simulink model "spikingTest"  (R2026b)
settings: Solver=FixedStepAuto  StopTime=1  FixedStep=0.001
libraries: simulink x1
settings Model: Creator=40129232  LastModifiedBy=Eoin
settings DataIOCC: ReturnWorkspaceOutputs=off
settings OptimizationCC: LifeSpan=inf
settings DebuggingCC: ArithmeticOperatorsInVariantConditions=warning  SFExecutionAtInitializationDiag=none
settings SFSimCC: CustomCodeUndefinedFunction=UseInterfaceOnly  SimUseLocalCustomCode=off
settings RTWCC: DLArmComputeVersion=19.05  RTWUseLocalCustomCode=off
settings CodeAppCC: StateflowObjectComments=on

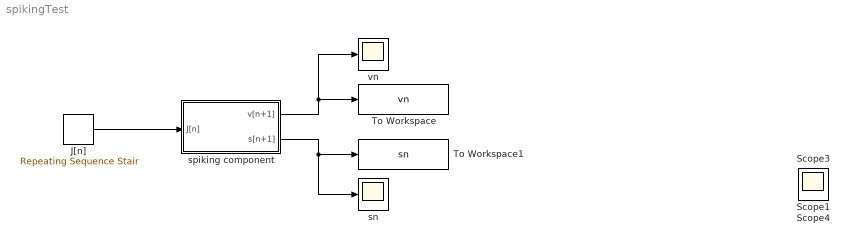
== system spikingTest ==
  J[n] : simulink/Sources/Repeating Sequence Stair  OutValues=[40.37, 52.35, 62.17, 70.19, 76.75].'  tsamp=-1  OutMin=[]  OutMax=[]  OutDataTypeStr=double  OutputDataTypeScalingMode=double  OutDataType=fixdt(0,8)  ConRadixGroup=Best Precision: Vector-wise  OutScaling=2^-12
  To Workspace : ToWorkspace  VariableName=vn  SaveFormat=Timeseries  SampleTime=-1
  To Workspace1 : ToWorkspace  VariableName=sn  SaveFormat=Timeseries  SampleTime=-1
  sn : Scope
      settings: ActiveDisplayYMinimum=-0.12499999999999997  ActiveDisplayYMaximum=1.125
  spiking component : Subsystem
  vn : Scope
      settings: ActiveDisplayYMinimum=-91.151379089259891  ActiveDisplayYMaximum=42.518602095331175  DataLoggingVariableName=ScopeData5
  Scope1 : Scope
      settings: ActiveDisplayYMinimum=-0.24987  ActiveDisplayYMaximum=2.24887
  Scope3 : Scope
      settings: ActiveDisplayYMinimum=-103.72127  ActiveDisplayYMaximum=38.33358  DataLoggingVariableName=ScopeData3
  Scope4 : Scope
      settings: ActiveDisplayYMinimum=-20.75486  ActiveDisplayYMaximum=56.79378  DataLoggingVariableName=ScopeData4
  wires:
  spiking component/1(v[n+1]) -> vn/1, To Workspace/1
  spiking component/2(s[n+1]) -> sn/1, To Workspace1/1
  J[n]/1 -> spiking component/1(J[n])

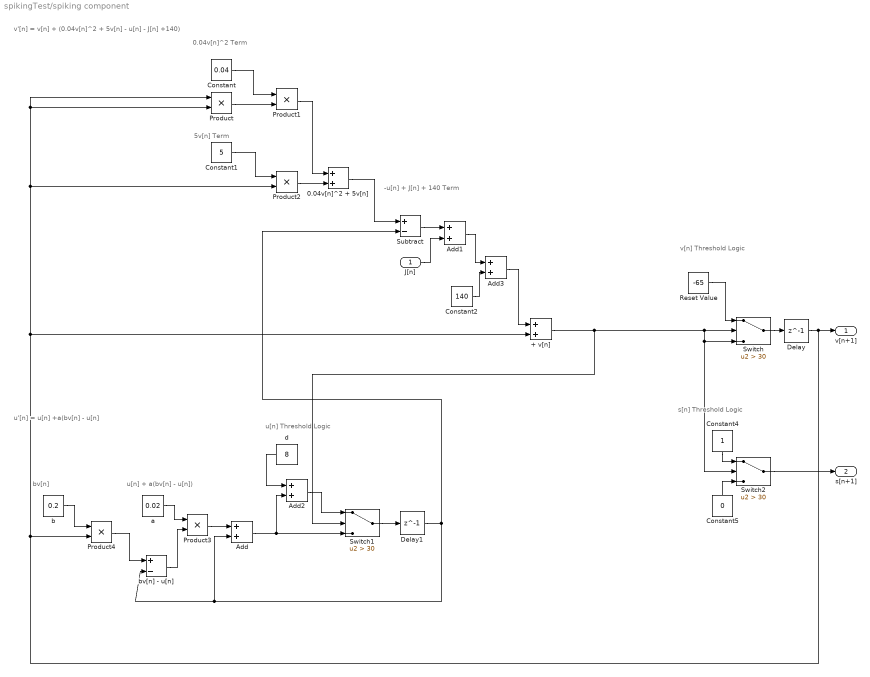
== system spikingTest/spiking component ==
  note: s[n] Threshold Logic
  note: v'[n] = v[n] + (0.04v[n]^2 + 5v[n] - u[n] - J[n] +140)
  note: u'[n] = u[n] +a(bv[n] - u[n]
  note: u[n] Threshold Logic
  note: u[n] + a(bv[n] - u[n])
  note: bv[n]
  note: v[n] Threshold Logic
  note: -u[n] + J[n] + 140 Term
  note: 5v[n] Term
  note: 0.04v[n]^2 Term
  J[n] : Inport  SampleTime=0.001
  + v[n] : Sum
  0.04v[n]^2 + 5v[n] : Sum
  Add{,1..3} (4 alike) : Sum
  Constant : Constant  Value=0.04
  Constant1 : Constant  Value=5
  Constant2 : Constant  Value=140
  Constant4 : Constant
  Constant5 : Constant  Value=0
  Delay : Delay  DelayLength=1  InitialCondition=-65
  Delay1 : Delay  DelayLength=1  InitialCondition=0
  Product{,1..4} (5 alike) : Product
  Reset Value : Constant  Value=-65
  Subtract : Sum  Inputs=+-
  Switch : Switch  Criteria=u2 > Threshold  Threshold=30  SaturateOnIntegerOverflow=off  InputSameDT=off
  Switch1 : Switch  Criteria=u2 > Threshold  Threshold=30  SaturateOnIntegerOverflow=off  InputSameDT=off
  Switch2 : Switch  Criteria=u2 > Threshold  Threshold=30  SaturateOnIntegerOverflow=off  InputSameDT=off
  a : Constant  Value=0.02
  b : Constant  Value=0.2
  bv[n] - u[n] : Sum  Inputs=+-
  d : Constant  Value=8
  v[n+1] : Outport  VectorParamsAs1DForOutWhenUnconnected=off
  s[n+1] : Outport  Port=2  VectorParamsAs1DForOutWhenUnconnected=off
  wires:
  Constant/1 -> Product1/1
  Product/1 -> Product1/2
  Product1/1 -> 0.04v[n]^2 + 5v[n]/1
  Product2/1 -> 0.04v[n]^2 + 5v[n]/2
  Constant1/1 -> Product2/1
  0.04v[n]^2 + 5v[n]/1 -> Subtract/1
  Subtract/1 -> Add1/1
  J[n]/1 -> Add1/2
  a/1 -> Product3/1
  b/1 -> Product4/1
  Product4/1 -> bv[n] - u[n]/1
  bv[n] - u[n]/1 -> Product3/2
  Product3/1 -> Add/1
  Add/1 -> Switch1/3, Add2/2
  Reset Value/1 -> Switch/1
  + v[n]/1 -> Switch/3, Switch2/2, Switch/2, Switch1/2
  Add2/1 -> Switch1/1
  d/1 -> Add2/1
  Constant4/1 -> Switch2/1
  Constant5/1 -> Switch2/3
  Switch2/1 -> s[n+1]/1
  Switch/1 -> Delay/1
  Switch1/1 -> Delay1/1
  Delay1/1 -> Add/2, bv[n] - u[n]/2, Subtract/2
  Add3/1 -> + v[n]/1
  Add1/1 -> Add3/1
  Constant2/1 -> Add3/2
  Delay/1 -> + v[n]/2, Product2/2, Product/2, Product/1, Product4/2, v[n+1]/1
